simulink model "EVChargingSimulation"  (R2026b)
settings: Solver=FixedStepDiscrete  StopTime=0
settings Model: Creator=aloytyno  LastModifiedBy=aloytyno

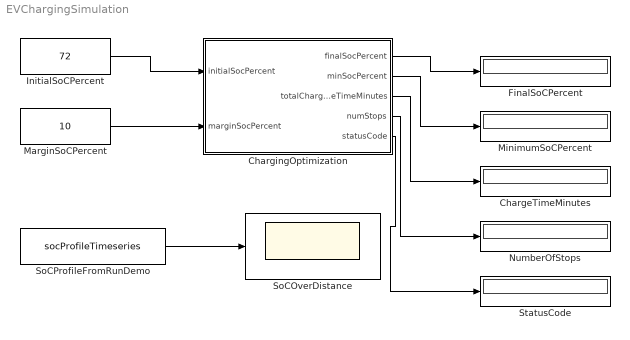
== system EVChargingSimulation ==
  ChargeTimeMinutes : Display
  ChargingOptimization : MATLAB Function  TreatAsAtomicUnit=on
  FinalSoCPercent : Display
  InitialSoCPercent : Constant  Value=72
  MarginSoCPercent : Constant  Value=10
  MinimumSoCPercent : Display
  NumberOfStops : Display
  SoCOverDistance : Scope
  SoCProfileFromRunDemo : FromWorkspace  VariableName=socProfileTimeseries
  StatusCode : Display
  wires:
  ChargingOptimization/1(finalSocPercent) -> FinalSoCPercent/1
  ChargingOptimization/2(minSocPercent) -> MinimumSoCPercent/1
  ChargingOptimization/3(totalChargeTimeMinutes) -> ChargeTimeMinutes/1
  ChargingOptimization/4(numStops) -> NumberOfStops/1
  ChargingOptimization/5(statusCode) -> StatusCode/1
  InitialSoCPercent/1 -> ChargingOptimization/1(initialSocPercent)
  MarginSoCPercent/1 -> ChargingOptimization/2(marginSocPercent)
  SoCProfileFromRunDemo/1 -> SoCOverDistance/1

== matlab function EVChargingSimulation/ChargingOptimization ==
  data: initialSocPercent input; finalSocPercent output; marginSocPercent input; minSocPercent output; totalChargeTimeMinutes output; numStops output; statusCode output
function [finalSocPercent, minSocPercent, totalChargeTimeMinutes, numStops, statusCode] = fcn(initialSocPercent, marginSocPercent)
%#codegen
coder.extrinsic('evcharge.simulinkEntryPoint');
finalSocPercent = 0;
minSocPercent = 0;
totalChargeTimeMinutes = 0;
numStops = 0;
statusCode = -1;
[finalSocPercent, minSocPercent, totalChargeTimeMinutes, numStops, statusCode] = evcharge.simulinkEntryPoint(initialSocPercent, marginSocPercent);
end
